simulink subsystem "Magnetorquer"  (R2024b)
settings: Solver=VariableStepAuto  StartTime=0.0  StopTime=10.0  RelTol=1e-3
model mask{R=0, k=0}
  mask prompts: R "Rotation matrix"; k "Scaling factor"
libraries: matrix_library x1
settings Model: Creator=marco  LastModifiedBy=ferru

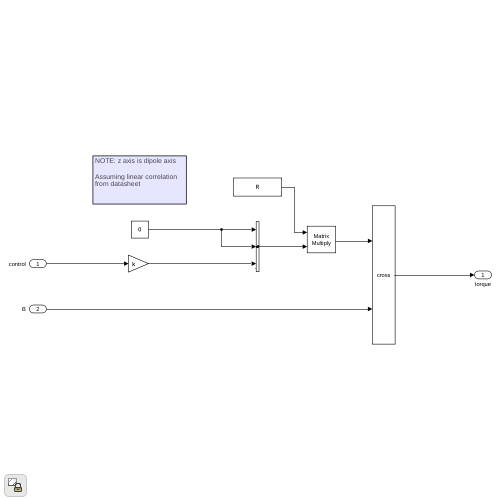
[thumbnail: Simulink's stored preview of the top-level diagram]
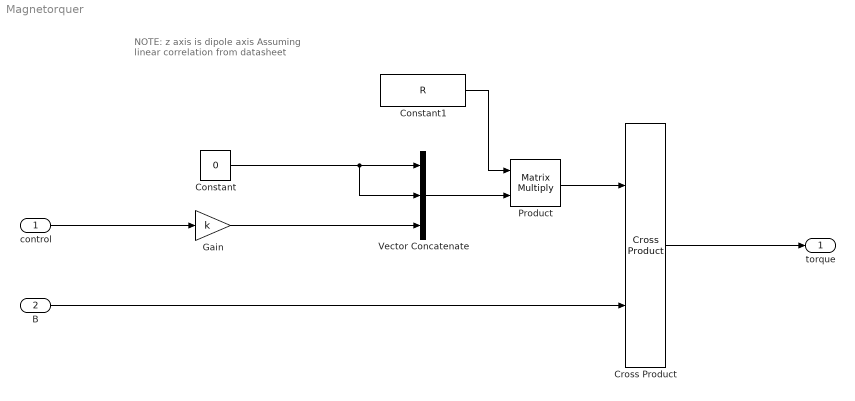
== system Magnetorquer ==
  note: NOTE: z axis is dipole axis
      |
      | Assuming linear correlation
      | from datasheet
  control : Inport
  B : Inport  Port=2
  Constant : Constant  Value=0
  Constant1 : Constant  Value=R  VectorParams1D=off
  Cross Product : matrix_library/Cross Product
  Gain : Gain  Gain=k
  Product : Product  Multiplication=Matrix(*)
  Vector Concatenate : Concatenate  NumInputs=3  Mode=Multidimensional array
  torque : Outport
  wires:
  control/1 -> Gain/1
  Constant/1 -> Vector Concatenate/1, Vector Concatenate/2
  Gain/1 -> Vector Concatenate/3
  Constant1/1 -> Product/1
  Vector Concatenate/1 -> Product/2
  Product/1 -> Cross Product/1
  B/1 -> Cross Product/2
  Cross Product/1 -> torque/1
